simulink model "day03_absolute_vs_delta"  (R2024a)
settings: Solver=ode45  StartTime=0.0  StopTime=4.0  MaxStep=0.01  RelTol=1e-8  AbsTol=1e-10
undefined symbols (not defined in the file or in its folder): g, m, T_total, U, v0, z0
settings Model: Creator=admin  LastModifiedBy=admin

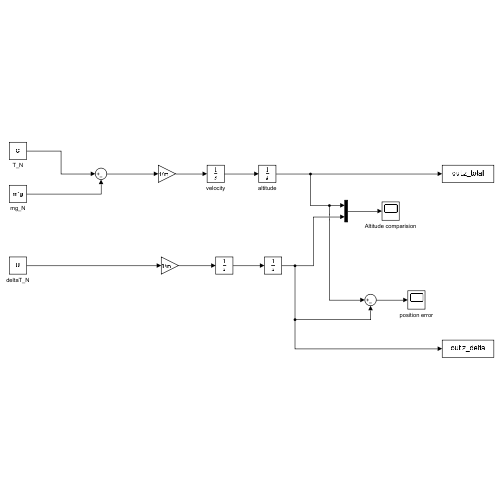
[thumbnail: Simulink's stored preview of the top-level diagram]
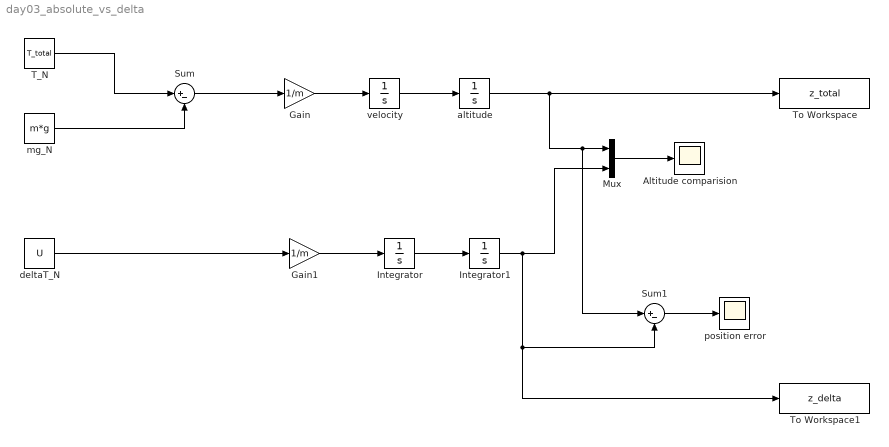
== system day03_absolute_vs_delta ==
  Altitude comparision : Scope
  Gain : Gain  Gain=1/m
  Gain1 : Gain  Gain=1/m
  Integrator : Integrator  InitialCondition=v0
  Integrator1 : Integrator  InitialCondition=z0
  Mux : Mux  Inputs=2
  Sum : Sum  Inputs=|+-
  Sum1 : Sum  Inputs=|+-
  T_N : Constant  Value=T_total
  To Workspace : ToWorkspace  VariableName=z_total  SaveFormat=Timeseries  SampleTime=-1
  To Workspace1 : ToWorkspace  VariableName=z_delta  SaveFormat=Timeseries  SampleTime=-1
  altitude : Integrator  InitialCondition=z0
  deltaT_N : Constant  Value=U
  mg_N : Constant  Value=m*g
  position error : Scope
  velocity : Integrator  InitialCondition=v0
  wires:
  T_N/1 -> Sum/1
  mg_N/1 -> Sum/2
  Sum/1 -> Gain/1
  Gain/1 -> velocity/1
  velocity/1 -> altitude/1
  deltaT_N/1 -> Gain1/1
  Gain1/1 -> Integrator/1
  Integrator/1 -> Integrator1/1
  altitude/1 -> To Workspace/1, Sum1/1, Mux/1
  Integrator1/1 -> To Workspace1/1, Sum1/2, Mux/2
  Mux/1 -> Altitude comparision/1
  Sum1/1 -> position error/1
